simulink model "ANN_MultiLoad_Generated"  (R2023a)
settings: Solver=VariableStepAuto  StartTime=0.0  StopTime=10.0  RelTol=1e-3
libraries: neural x25
settings Model: Creator=Sooraj Mohan  LastModifiedBy=Sooraj Mohan

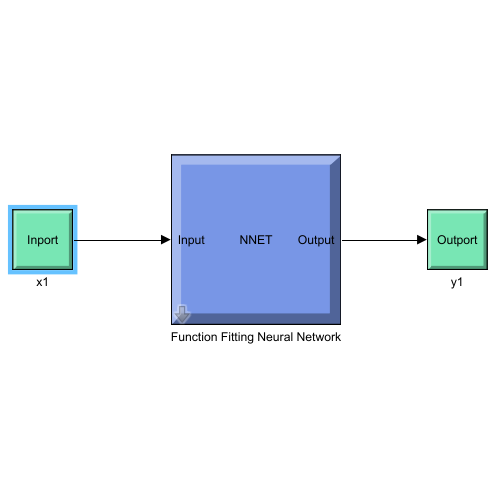
[thumbnail: Simulink's stored preview of the top-level diagram]
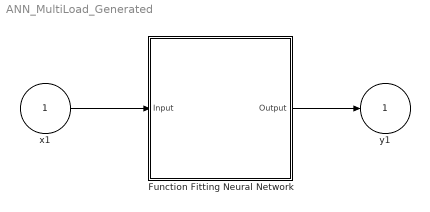
== system ANN_MultiLoad_Generated ==
  x1 : Inport  PortDimensions=3
      mask Display: e = 0.06;c1 = [120 230 180]/255;c2 = ([120 230 180]+0)/(256+128);c3 = ([120 230 180]+128)/(256+128);patch([0 1 1 0],[0 0 1 1],c1);patch([0 1 1 1-e 1-e 0+e],[0 0 1 1-e 0+e 0+e],c2);patch([0 0 1 1-e 0+e 0+e],[0 1 1 1-e 1-e 0+e],c3);plot([0 1 1 0 0],[0 0 1 1 0]);disp('Inport');
  Function Fitting Neural Network : Subsystem
      mask help: Function Fitting Neural Network
      mask Display: e = 0.06;c1 = [120 150 230]/255;c2 = ([120 150 230]+0)/383;c3 = ([120 150 230]+128)/383;patch([0 1 1 0],[0 0 1 1],c1);patch([0 1 1 1-e 1-e 0+e],[0 0 1 1-e 0+e 0+e],c2);patch([0 0 1 1-e 0+e 0+e],[0 1 1 1-e 1-e 0+e],c3);plot([0 1 1 0 0],[0 0 1 1 0]);fprintf('NNET');port_label('input',1,' Input');port_label('output',1,'Output ');
  y1 : Outport  PortDimensions=1
      mask Display: e = 0.06;c1 = [120 230 180]/255;c2 = ([120 230 180]+0)/(256+128);c3 = ([120 230 180]+128)/(256+128);patch([0 1 1 0],[0 0 1 1],c1);patch([0 1 1 1-e 1-e 0+e],[0 0 1 1-e 0+e 0+e],c2);patch([0 0 1 1-e 0+e 0+e],[0 1 1 1-e 1-e 0+e],c3);plot([0 1 1 0 0],[0 0 1 1 0]);disp('Outport');
  wires:
  x1/1 -> Function Fitting Neural Network/1(Input)
  Function Fitting Neural Network/1(Output) -> y1/1

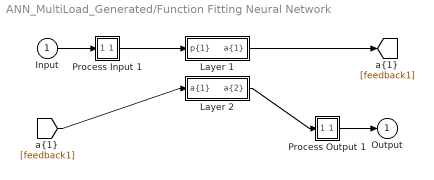
== system ANN_MultiLoad_Generated/Function Fitting Neural Network ==
  Input : Inport  PortDimensions=3
      mask Display: e = 0.06;c1 = [120 230 180]/255;c2 = ([120 230 180]+0)/(256+128);c3 = ([120 230 180]+128)/(256+128);patch([0 1 1 0],[0 0 1 1],c1);patch([0 1 1 1-e 1-e 0+e],[0 0 1 1-e 0+e 0+e],c2);patch([0 0 1 1-e 0+e 0+e],[0 1 1 1-e 1-e 0+e],c3);plot([0 1 1 0 0],[0 0 1 1 0]);
  Layer 1 : Subsystem
      mask Display: e = 0.06;c1 = [120 150 230]/255;c2 = ([120 150 230]+0)/383;c3 = ([120 150 230]+128)/383;patch([0 1 1 0],[0 0 1 1],c1);patch([0 1 1 1-e 1-e 0+e],[0 0 1 1-e 0+e 0+e],c2);patch([0 0 1 1-e 0+e 0+e],[0 1 1 1-e 1-e 0+e],c3);plot([0 1 1 0 0],[0 0 1 1 0]);
  Layer 2 : Subsystem
      mask Display: e = 0.06;c1 = [120 150 230]/255;c2 = ([120 150 230]+0)/383;c3 = ([120 150 230]+128)/383;patch([0 1 1 0],[0 0 1 1],c1);patch([0 1 1 1-e 1-e 0+e],[0 0 1 1-e 0+e 0+e],c2);patch([0 0 1 1-e 0+e 0+e],[0 1 1 1-e 1-e 0+e],c3);plot([0 1 1 0 0],[0 0 1 1 0]);
  Process Input 1 : Subsystem
      mask Display: e = 0.06;c1 = [120 150 230]/255;c2 = ([120 150 230]+0)/383;c3 = ([120 150 230]+128)/383;patch([0 1 1 0],[0 0 1 1],c1);patch([0 1 1 1-e 1-e 0+e],[0 0 1 1-e 0+e 0+e],c2);patch([0 0 1 1-e 0+e 0+e],[0 1 1 1-e 1-e 0+e],c3);plot([0 1 1 0 0],[0 0 1 1 0]);
  Process Output 1 : Subsystem
      mask Display: e = 0.06;c1 = [120 150 230]/255;c2 = ([120 150 230]+0)/383;c3 = ([120 150 230]+128)/383;patch([0 1 1 0],[0 0 1 1],c1);patch([0 1 1 1-e 1-e 0+e],[0 0 1 1-e 0+e 0+e],c2);patch([0 0 1 1-e 0+e 0+e],[0 1 1 1-e 1-e 0+e],c3);plot([0 1 1 0 0],[0 0 1 1 0]);
  Output : Outport  InitialOutput=0
      mask Display: e = 0.06;c1 = [120 230 180]/255;c2 = ([120 230 180]+0)/(256+128);c3 = ([120 230 180]+128)/(256+128);patch([0 1 1 0],[0 0 1 1],c1);patch([0 1 1 1-e 1-e 0+e],[0 0 1 1-e 0+e 0+e],c2);patch([0 0 1 1-e 0+e 0+e],[0 1 1 1-e 1-e 0+e],c3);plot([0 1 1 0 0],[0 0 1 1 0]);
  wires:
  Input/1 -> Process Input 1/1(x)
  Process Output 1/1(y) -> Output/1
  Process Input 1/1(p) -> Layer 1/1("p{1}")
  Layer 1/1("a{1}") -> [feedback1]
  [feedback1] -> Layer 2/1("a{1} ")
  Layer 2/1("a{2}") -> Process Output 1/1(a)

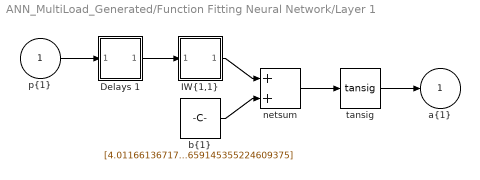
== system ANN_MultiLoad_Generated/Function Fitting Neural Network/Layer 1 ==
  "p{1}" : Inport  PortDimensions=3
      mask Display: e = 0.06;c1 = [120 230 180]/255;c2 = ([120 230 180]+0)/(256+128);c3 = ([120 230 180]+128)/(256+128);patch([0 1 1 0],[0 0 1 1],c1);patch([0 1 1 1-e 1-e 0+e],[0 0 1 1-e 0+e 0+e],c2);patch([0 0 1 1-e 0+e 0+e],[0 1 1 1-e 1-e 0+e],c3);plot([0 1 1 0 0],[0 0 1 1 0]);
  Delays 1 : Subsystem
      mask Display: e = 0.06;c1 = [120 150 230]/255;c2 = ([120 150 230]+0)/383;c3 = ([120 150 230]+128)/383;patch([0 1 1 0],[0 0 1 1],c1);patch([0 1 1 1-e 1-e 0+e],[0 0 1 1-e 0+e 0+e],c2);patch([0 0 1 1-e 0+e 0+e],[0 1 1 1-e 1-e 0+e],c3);plot([0 1 1 0 0],[0 0 1 1 0]);disp('0');
  "IW{1,1}" : Subsystem
      mask Display: e = 0.06;c1 = [120 150 230]/255;c2 = ([120 150 230]+0)/383;c3 = ([120 150 230]+128)/383;patch([0 1 1 0],[0 0 1 1],c1);patch([0 1 1 1-e 1-e 0+e],[0 0 1 1-e 0+e 0+e],c2);patch([0 0 1 1-e 0+e 0+e],[0 1 1 1-e 1-e 0+e],c3);plot([0 1 1 0 0],[0 0 1 1 0]);disp('W');
  "b{1}" : Constant  Value=[4.01166136717708976533458553603850305080413818359375;3.425657584804036925874015651061199605464935302734375;2.945133302338741376757980106049217283725738525390625;2.487472514834082826240546637563966214656829833984375;-2.198586640079299936445522689609788358211517333984375;-1.6511881060762032547017952310852706432342529296875;-0.9569310901758696363827993991435505449771881103515625;0.80526211729380448023363214815617538988590240478515625;0.63594565591895457767890320610604248940944671630859375;0.5017187841956556315636817089398391544818878173828125;0.09104143474311969519430220998401637189090251922607421875;-0.74022312093395414844820834332494996488094329833984375;-1.012970720944128544260820490308105945587158203125;-1.3663031771011218129530107034952379763126373291015625;1.8030354517322588758787560436758212745189666748046875;2.208400225146431861134033169946633279323577880859375;2.71632750565131431130794226191937923431396484375;-3.080179604871890131079226193833164870738983154296875;3.44002398306910261993607491604052484035491943359375;-3.78824406270324853807096587843261659145355224609375]
      mask Display: e = 0.06;c1 = [120 150 230]/255;c2 = ([120 150 230]+0)/383;c3 = ([120 150 230]+128)/383;patch([0 1 1 0],[0 0 1 1],c1);patch([0 1 1 1-e 1-e 0+e],[0 0 1 1-e 0+e 0+e],c2);patch([0 0 1 1-e 0+e 0+e],[0 1 1 1-e 1-e 0+e],c3);plot([0 1 1 0 0],[0 0 1 1 0]);disp('b');
  netsum : Sum  Inputs=2  InputSameDT=on  SaturateOnIntegerOverflow=on  OutDataTypeStr=Inherit: Same as first input
      mask Display: e = 0.06;c1 = [120 150 230]/255;c2 = ([120 150 230]+0)/383;c3 = ([120 150 230]+128)/383;patch([0 1 1 0],[0 0 1 1],c1);patch([0 1 1 1-e 1-e 0+e],[0 0 1 1-e 0+e 0+e],c2);patch([0 0 1 1-e 0+e 0+e],[0 1 1 1-e 1-e 0+e],c3);plot([0 1 1 0 0],[0 0 1 1 0]);disp('+');
  tansig : neural/Transfer Functions/tansig
  "a{1}" : Outport  InitialOutput=[0;0;0;0;0;0;0;0;0;0;0;0;0;0;0;0;0;0;0;0]
      mask Display: e = 0.06;c1 = [120 230 180]/255;c2 = ([120 230 180]+0)/(256+128);c3 = ([120 230 180]+128)/(256+128);patch([0 1 1 0],[0 0 1 1],c1);patch([0 1 1 1-e 1-e 0+e],[0 0 1 1-e 0+e 0+e],c2);patch([0 0 1 1-e 0+e 0+e],[0 1 1 1-e 1-e 0+e],c3);plot([0 1 1 0 0],[0 0 1 1 0]);
  wires:
  "p{1}"/1 -> Delays 1/1("p{1}")
  Delays 1/1("pd{1,1}") -> "IW{1,1}"/1("pd{1,1}")
  "IW{1,1}"/1("iz{1,1}") -> netsum/1
  "b{1}"/1 -> netsum/2
  netsum/1 -> tansig/1
  tansig/1 -> "a{1}"/1

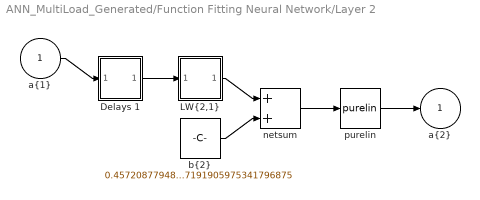
== system ANN_MultiLoad_Generated/Function Fitting Neural Network/Layer 2 ==
  "a{1} " : Inport  PortDimensions=20
      mask Display: e = 0.06;c1 = [120 230 180]/255;c2 = ([120 230 180]+0)/(256+128);c3 = ([120 230 180]+128)/(256+128);patch([0 1 1 0],[0 0 1 1],c1);patch([0 1 1 1-e 1-e 0+e],[0 0 1 1-e 0+e 0+e],c2);patch([0 0 1 1-e 0+e 0+e],[0 1 1 1-e 1-e 0+e],c3);plot([0 1 1 0 0],[0 0 1 1 0]);
  Delays 1 : Subsystem
      mask Display: e = 0.06;c1 = [120 150 230]/255;c2 = ([120 150 230]+0)/383;c3 = ([120 150 230]+128)/383;patch([0 1 1 0],[0 0 1 1],c1);patch([0 1 1 1-e 1-e 0+e],[0 0 1 1-e 0+e 0+e],c2);patch([0 0 1 1-e 0+e 0+e],[0 1 1 1-e 1-e 0+e],c3);plot([0 1 1 0 0],[0 0 1 1 0]);disp('0');
  "LW{2,1}" : Subsystem
      mask Display: e = 0.06;c1 = [120 150 230]/255;c2 = ([120 150 230]+0)/383;c3 = ([120 150 230]+128)/383;patch([0 1 1 0],[0 0 1 1],c1);patch([0 1 1 1-e 1-e 0+e],[0 0 1 1-e 0+e 0+e],c2);patch([0 0 1 1-e 0+e 0+e],[0 1 1 1-e 1-e 0+e],c3);plot([0 1 1 0 0],[0 0 1 1 0]);disp('W');
  "b{2}" : Constant  Value=0.4572087794873869182055159399169497191905975341796875
      mask Display: e = 0.06;c1 = [120 150 230]/255;c2 = ([120 150 230]+0)/383;c3 = ([120 150 230]+128)/383;patch([0 1 1 0],[0 0 1 1],c1);patch([0 1 1 1-e 1-e 0+e],[0 0 1 1-e 0+e 0+e],c2);patch([0 0 1 1-e 0+e 0+e],[0 1 1 1-e 1-e 0+e],c3);plot([0 1 1 0 0],[0 0 1 1 0]);disp('b');
  netsum : Sum  Inputs=2  InputSameDT=on  SaturateOnIntegerOverflow=on  OutDataTypeStr=Inherit: Same as first input
      mask Display: e = 0.06;c1 = [120 150 230]/255;c2 = ([120 150 230]+0)/383;c3 = ([120 150 230]+128)/383;patch([0 1 1 0],[0 0 1 1],c1);patch([0 1 1 1-e 1-e 0+e],[0 0 1 1-e 0+e 0+e],c2);patch([0 0 1 1-e 0+e 0+e],[0 1 1 1-e 1-e 0+e],c3);plot([0 1 1 0 0],[0 0 1 1 0]);disp('+');
  purelin : neural/Transfer Functions/purelin
  "a{2}" : Outport  InitialOutput=0
      mask Display: e = 0.06;c1 = [120 230 180]/255;c2 = ([120 230 180]+0)/(256+128);c3 = ([120 230 180]+128)/(256+128);patch([0 1 1 0],[0 0 1 1],c1);patch([0 1 1 1-e 1-e 0+e],[0 0 1 1-e 0+e 0+e],c2);patch([0 0 1 1-e 0+e 0+e],[0 1 1 1-e 1-e 0+e],c3);plot([0 1 1 0 0],[0 0 1 1 0]);
  wires:
  "a{1} "/1 -> Delays 1/1("p{2}")
  Delays 1/1("pd{2,1}") -> "LW{2,1}"/1("ad{2,1}")
  "LW{2,1}"/1("lz{2,1}") -> netsum/1
  "b{2}"/1 -> netsum/2
  netsum/1 -> purelin/1
  purelin/1 -> "a{2}"/1

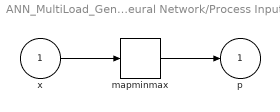
== system ANN_MultiLoad_Generated/Function Fitting Neural Network/Process Input 1 ==
  x : Inport  PortDimensions=3
      mask Display: e = 0.06;c1 = [120 230 180]/255;c2 = ([120 230 180]+0)/(256+128);c3 = ([120 230 180]+128)/(256+128);patch([0 1 1 0],[0 0 1 1],c1);patch([0 1 1 1-e 1-e 0+e],[0 0 1 1-e 0+e 0+e],c2);patch([0 0 1 1-e 0+e 0+e],[0 1 1 1-e 1-e 0+e],c3);plot([0 1 1 0 0],[0 0 1 1 0]);
  mapminmax : neural/Processing Functions/mapminmax  xmin=[-5.41533881963086471955648448784;-353.856954219733665922831278294;400.000000000000056843418860808]  xmax=[5.40694529891772912577607712592;355.597694951485948422487126663;400.000000000000113686837721616]  ymin=-1  ymax=1
  p : Outport  PortDimensions=3
      mask Display: e = 0.06;c1 = [120 230 180]/255;c2 = ([120 230 180]+0)/(256+128);c3 = ([120 230 180]+128)/(256+128);patch([0 1 1 0],[0 0 1 1],c1);patch([0 1 1 1-e 1-e 0+e],[0 0 1 1-e 0+e 0+e],c2);patch([0 0 1 1-e 0+e 0+e],[0 1 1 1-e 1-e 0+e],c3);plot([0 1 1 0 0],[0 0 1 1 0]);
  wires:
  x/1 -> mapminmax/1
  mapminmax/1 -> p/1

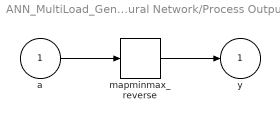
== system ANN_MultiLoad_Generated/Function Fitting Neural Network/Process Output 1 ==
  a : Inport  PortDimensions=1
      mask Display: e = 0.06;c1 = [120 230 180]/255;c2 = ([120 230 180]+0)/(256+128);c3 = ([120 230 180]+128)/(256+128);patch([0 1 1 0],[0 0 1 1],c1);patch([0 1 1 1-e 1-e 0+e],[0 0 1 1-e 0+e 0+e],c2);patch([0 0 1 1-e 0+e 0+e],[0 1 1 1-e 1-e 0+e],c3);plot([0 1 1 0 0],[0 0 1 1 0]);
  mapminmax_reverse : neural/Processing Functions/mapminmax_reverse  xmin=-85.1861603832918632406290271319  xmax=79.5292501519603263204771792516  ymin=-1  ymax=1
  y : Outport  PortDimensions=1
      mask Display: e = 0.06;c1 = [120 230 180]/255;c2 = ([120 230 180]+0)/(256+128);c3 = ([120 230 180]+128)/(256+128);patch([0 1 1 0],[0 0 1 1],c1);patch([0 1 1 1-e 1-e 0+e],[0 0 1 1-e 0+e 0+e],c2);patch([0 0 1 1-e 0+e 0+e],[0 1 1 1-e 1-e 0+e],c3);plot([0 1 1 0 0],[0 0 1 1 0]);
  wires:
  a/1 -> mapminmax_reverse/1
  mapminmax_reverse/1 -> y/1

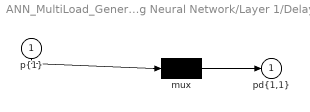
== system ANN_MultiLoad_Generated/Function Fitting Neural Network/Layer 1/Delays 1 ==
  "p{1}" : Inport  PortDimensions=3
      mask Display: e = 0.06;c1 = [120 230 180]/255;c2 = ([120 230 180]+0)/(256+128);c3 = ([120 230 180]+128)/(256+128);patch([0 1 1 0],[0 0 1 1],c1);patch([0 1 1 1-e 1-e 0+e],[0 0 1 1-e 0+e 0+e],c2);patch([0 0 1 1-e 0+e 0+e],[0 1 1 1-e 1-e 0+e],c3);plot([0 1 1 0 0],[0 0 1 1 0]);
  mux : Mux  Inputs=1
      mask Display: e = 0.06;c1 = [120 150 230]/255;c2 = ([120 150 230]+0)/383;c3 = ([120 150 230]+128)/383;patch([0 1 1 0],[0 0 1 1],c1);patch([0 1 1 1-e 1-e 0+e],[0 0 1 1-e 0+e 0+e],c2);patch([0 0 1 1-e 0+e 0+e],[0 1 1 1-e 1-e 0+e],c3);plot([0 1 1 0 0],[0 0 1 1 0]);disp('Mux')
  "pd{1,1}" : Outport
      mask Display: e = 0.06;c1 = [120 230 180]/255;c2 = ([120 230 180]+0)/(256+128);c3 = ([120 230 180]+128)/(256+128);patch([0 1 1 0],[0 0 1 1],c1);patch([0 1 1 1-e 1-e 0+e],[0 0 1 1-e 0+e 0+e],c2);patch([0 0 1 1-e 0+e 0+e],[0 1 1 1-e 1-e 0+e],c3);plot([0 1 1 0 0],[0 0 1 1 0]);
  wires:
  "p{1}"/1 -> mux/1
  mux/1 -> "pd{1,1}"/1

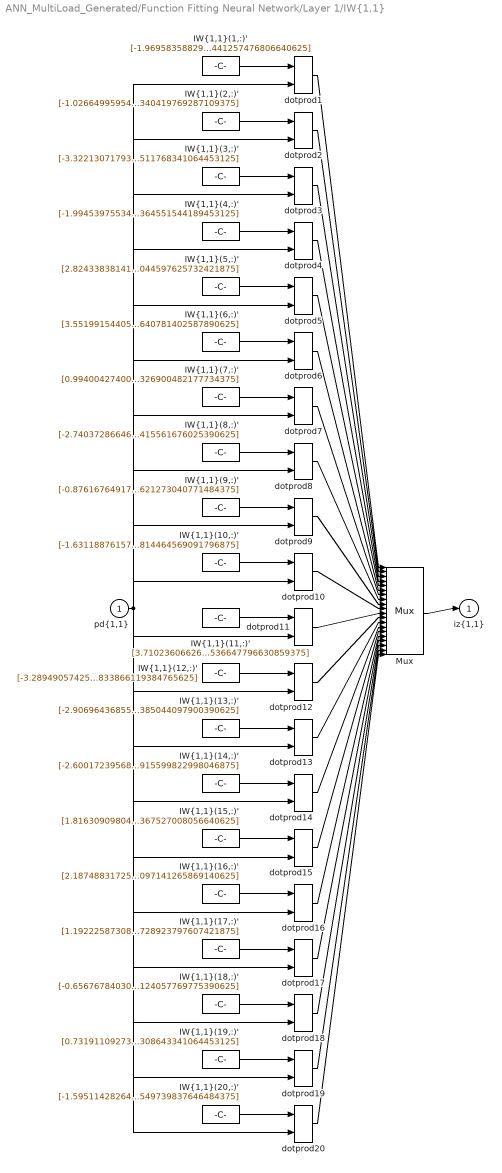
== system ANN_MultiLoad_Generated/Function Fitting Neural Network/Layer 1/IW{1,1} ==
  "pd{1,1}" : Inport  PortDimensions=3
      mask Display: e = 0.06;c1 = [120 230 180]/255;c2 = ([120 230 180]+0)/(256+128);c3 = ([120 230 180]+128)/(256+128);patch([0 1 1 0],[0 0 1 1],c1);patch([0 1 1 1-e 1-e 0+e],[0 0 1 1-e 0+e 0+e],c2);patch([0 0 1 1-e 0+e 0+e],[0 1 1 1-e 1-e 0+e],c3);plot([0 1 1 0 0],[0 0 1 1 0]);
  "IW{1,1}(1,:)'" : Constant  Value=[-1.96958358829980539894677349366247653961181640625;1.918521251483812140037343851872719824314117431640625;2.29210042612150033392026671208441257476806640625]
      mask Display: e = 0.06;c1 = [120 150 230]/255;c2 = ([120 150 230]+0)/383;c3 = ([120 150 230]+128)/383;patch([0 1 1 0],[0 0 1 1],c1);patch([0 1 1 1-e 1-e 0+e],[0 0 1 1-e 0+e 0+e],c2);patch([0 0 1 1-e 0+e 0+e],[0 1 1 1-e 1-e 0+e],c3);plot([0 1 1 0 0],[0 0 1 1 0]);disp('Weights');
  "IW{1,1}(10,:)'" : Constant  Value=[-1.6311887615787288297042323392815887928009033203125;2.51590885704565447866798422182910144329071044921875;-2.3411727844511727170129233854822814464569091796875]
      mask Display: e = 0.06;c1 = [120 150 230]/255;c2 = ([120 150 230]+0)/383;c3 = ([120 150 230]+128)/383;patch([0 1 1 0],[0 0 1 1],c1);patch([0 1 1 1-e 1-e 0+e],[0 0 1 1-e 0+e 0+e],c2);patch([0 0 1 1-e 0+e 0+e],[0 1 1 1-e 1-e 0+e],c3);plot([0 1 1 0 0],[0 0 1 1 0]);disp('Weights');
  "IW{1,1}(11,:)'" : Constant  Value=[3.71023606626158386490033080917783081531524658203125;-0.5979197475541944140076111580128781497478485107421875;-0.2575045382185476849912220131955109536647796630859375]
      mask Display: e = 0.06;c1 = [120 150 230]/255;c2 = ([120 150 230]+0)/383;c3 = ([120 150 230]+128)/383;patch([0 1 1 0],[0 0 1 1],c1);patch([0 1 1 1-e 1-e 0+e],[0 0 1 1-e 0+e 0+e],c2);patch([0 0 1 1-e 0+e 0+e],[0 1 1 1-e 1-e 0+e],c3);plot([0 1 1 0 0],[0 0 1 1 0]);disp('Weights');
  "IW{1,1}(12,:)'" : Constant  Value=[-3.289490574255142352200209643342532217502593994140625;-0.5469995320266207716741746480693109333515167236328125;-1.6949446183999461457148072440759278833866119384765625]
      mask Display: e = 0.06;c1 = [120 150 230]/255;c2 = ([120 150 230]+0)/383;c3 = ([120 150 230]+128)/383;patch([0 1 1 0],[0 0 1 1],c1);patch([0 1 1 1-e 1-e 0+e],[0 0 1 1-e 0+e 0+e],c2);patch([0 0 1 1-e 0+e 0+e],[0 1 1 1-e 1-e 0+e],c3);plot([0 1 1 0 0],[0 0 1 1 0]);disp('Weights');
  "IW{1,1}(13,:)'" : Constant  Value=[-2.906964368554389555043826476321555674076080322265625;-0.5995612852190375097194419140578247606754302978515625;2.299154545812025052242688616388477385044097900390625]
      mask Display: e = 0.06;c1 = [120 150 230]/255;c2 = ([120 150 230]+0)/383;c3 = ([120 150 230]+128)/383;patch([0 1 1 0],[0 0 1 1],c1);patch([0 1 1 1-e 1-e 0+e],[0 0 1 1-e 0+e 0+e],c2);patch([0 0 1 1-e 0+e 0+e],[0 1 1 1-e 1-e 0+e],c3);plot([0 1 1 0 0],[0 0 1 1 0]);disp('Weights');
  "IW{1,1}(14,:)'" : Constant  Value=[-2.60017239568569547003562547615729272365570068359375;-1.2913554073851207792955619879649020731449127197265625;-2.40019667610683296032902944716624915599822998046875]
      mask Display: e = 0.06;c1 = [120 150 230]/255;c2 = ([120 150 230]+0)/383;c3 = ([120 150 230]+128)/383;patch([0 1 1 0],[0 0 1 1],c1);patch([0 1 1 1-e 1-e 0+e],[0 0 1 1-e 0+e 0+e],c2);patch([0 0 1 1-e 0+e 0+e],[0 1 1 1-e 1-e 0+e],c3);plot([0 1 1 0 0],[0 0 1 1 0]);disp('Weights');
  "IW{1,1}(15,:)'" : Constant  Value=[1.8163090980494087656182955470285378396511077880859375;0.1027208588357631235954414705702220089733600616455078125;-3.33268860031713476388404160388745367527008056640625]
      mask Display: e = 0.06;c1 = [120 150 230]/255;c2 = ([120 150 230]+0)/383;c3 = ([120 150 230]+128)/383;patch([0 1 1 0],[0 0 1 1],c1);patch([0 1 1 1-e 1-e 0+e],[0 0 1 1-e 0+e 0+e],c2);patch([0 0 1 1-e 0+e 0+e],[0 1 1 1-e 1-e 0+e],c3);plot([0 1 1 0 0],[0 0 1 1 0]);disp('Weights');
  "IW{1,1}(16,:)'" : Constant  Value=[2.18748831725833259298497068812139332294464111328125;0.10090970176754243681216394179500639438629150390625;-3.0963102908207762453685063519515097141265869140625]
      mask Display: e = 0.06;c1 = [120 150 230]/255;c2 = ([120 150 230]+0)/383;c3 = ([120 150 230]+128)/383;patch([0 1 1 0],[0 0 1 1],c1);patch([0 1 1 1-e 1-e 0+e],[0 0 1 1-e 0+e 0+e],c2);patch([0 0 1 1-e 0+e 0+e],[0 1 1 1-e 1-e 0+e],c3);plot([0 1 1 0 0],[0 0 1 1 0]);disp('Weights');
  "IW{1,1}(17,:)'" : Constant  Value=[1.19222587308537786299211802543140947818756103515625;2.60340339909535156692754753748886287212371826171875;-2.433568542835882198005492682568728923797607421875]
      mask Display: e = 0.06;c1 = [120 150 230]/255;c2 = ([120 150 230]+0)/383;c3 = ([120 150 230]+128)/383;patch([0 1 1 0],[0 0 1 1],c1);patch([0 1 1 1-e 1-e 0+e],[0 0 1 1-e 0+e 0+e],c2);patch([0 0 1 1-e 0+e 0+e],[0 1 1 1-e 1-e 0+e],c3);plot([0 1 1 0 0],[0 0 1 1 0]);disp('Weights');
  "IW{1,1}(18,:)'" : Constant  Value=[-0.65676784030766033328774256005999632179737091064453125;3.60318263358925516826047896756790578365325927734375;-0.7192382964292927116645159912877716124057769775390625]
      mask Display: e = 0.06;c1 = [120 150 230]/255;c2 = ([120 150 230]+0)/383;c3 = ([120 150 230]+128)/383;patch([0 1 1 0],[0 0 1 1],c1);patch([0 1 1 1-e 1-e 0+e],[0 0 1 1-e 0+e 0+e],c2);patch([0 0 1 1-e 0+e 0+e],[0 1 1 1-e 1-e 0+e],c3);plot([0 1 1 0 0],[0 0 1 1 0]);disp('Weights');
  "IW{1,1}(19,:)'" : Constant  Value=[0.73191109273039334226496066548861563205718994140625;2.25441141521850685336403330438770353794097900390625;-2.93828389411340840098318949458189308643341064453125]
      mask Display: e = 0.06;c1 = [120 150 230]/255;c2 = ([120 150 230]+0)/383;c3 = ([120 150 230]+128)/383;patch([0 1 1 0],[0 0 1 1],c1);patch([0 1 1 1-e 1-e 0+e],[0 0 1 1-e 0+e 0+e],c2);patch([0 0 1 1-e 0+e 0+e],[0 1 1 1-e 1-e 0+e],c3);plot([0 1 1 0 0],[0 0 1 1 0]);disp('Weights');
  "IW{1,1}(2,:)'" : Constant  Value=[-1.0266499595402311939551509567536413669586181640625;-3.750127303457734040392779206740669906139373779296875;0.3558927058893279760098948827362619340419769287109375]
      mask Display: e = 0.06;c1 = [120 150 230]/255;c2 = ([120 150 230]+0)/383;c3 = ([120 150 230]+128)/383;patch([0 1 1 0],[0 0 1 1],c1);patch([0 1 1 1-e 1-e 0+e],[0 0 1 1-e 0+e 0+e],c2);patch([0 0 1 1-e 0+e 0+e],[0 1 1 1-e 1-e 0+e],c3);plot([0 1 1 0 0],[0 0 1 1 0]);disp('Weights');
  "IW{1,1}(20,:)'" : Constant  Value=[-1.59511428264959054246219238848425447940826416015625;-0.950804370965463885312374259228818118572235107421875;3.32740866167332427494329749606549739837646484375]
      mask Display: e = 0.06;c1 = [120 150 230]/255;c2 = ([120 150 230]+0)/383;c3 = ([120 150 230]+128)/383;patch([0 1 1 0],[0 0 1 1],c1);patch([0 1 1 1-e 1-e 0+e],[0 0 1 1-e 0+e 0+e],c2);patch([0 0 1 1-e 0+e 0+e],[0 1 1 1-e 1-e 0+e],c3);plot([0 1 1 0 0],[0 0 1 1 0]);disp('Weights');
  "IW{1,1}(3,:)'" : Constant  Value=[-3.3221307179311754254058541846461594104766845703125;1.470211676342646267556801831233315169811248779296875;-1.160407496704341401283500090357847511768341064453125]
      mask Display: e = 0.06;c1 = [120 150 230]/255;c2 = ([120 150 230]+0)/383;c3 = ([120 150 230]+128)/383;patch([0 1 1 0],[0 0 1 1],c1);patch([0 1 1 1-e 1-e 0+e],[0 0 1 1-e 0+e 0+e],c2);patch([0 0 1 1-e 0+e 0+e],[0 1 1 1-e 1-e 0+e],c3);plot([0 1 1 0 0],[0 0 1 1 0]);disp('Weights');
  "IW{1,1}(4,:)'" : Constant  Value=[-1.9945397553436254867165189352817833423614501953125;-1.2838945124631575556151119599235244095325469970703125;2.661710597616452123048702560481615364551544189453125]
      mask Display: e = 0.06;c1 = [120 150 230]/255;c2 = ([120 150 230]+0)/383;c3 = ([120 150 230]+128)/383;patch([0 1 1 0],[0 0 1 1],c1);patch([0 1 1 1-e 1-e 0+e],[0 0 1 1-e 0+e 0+e],c2);patch([0 0 1 1-e 0+e 0+e],[0 1 1 1-e 1-e 0+e],c3);plot([0 1 1 0 0],[0 0 1 1 0]);disp('Weights');
  "IW{1,1}(5,:)'" : Constant  Value=[2.824338381411645837459900576504878699779510498046875;-0.8391692684293392545669121318496763706207275390625;2.400397949837205668899287047679536044597625732421875]
      mask Display: e = 0.06;c1 = [120 150 230]/255;c2 = ([120 150 230]+0)/383;c3 = ([120 150 230]+128)/383;patch([0 1 1 0],[0 0 1 1],c1);patch([0 1 1 1-e 1-e 0+e],[0 0 1 1-e 0+e 0+e],c2);patch([0 0 1 1-e 0+e 0+e],[0 1 1 1-e 1-e 0+e],c3);plot([0 1 1 0 0],[0 0 1 1 0]);disp('Weights');
  "IW{1,1}(6,:)'" : Constant  Value=[3.551991544055625116271812657942064106464385986328125;1.1022017018245733321890611478011123836040496826171875;0.25867677418343115736121262671076692640781402587890625]
      mask Display: e = 0.06;c1 = [120 150 230]/255;c2 = ([120 150 230]+0)/383;c3 = ([120 150 230]+128)/383;patch([0 1 1 0],[0 0 1 1],c1);patch([0 1 1 1-e 1-e 0+e],[0 0 1 1-e 0+e 0+e],c2);patch([0 0 1 1-e 0+e 0+e],[0 1 1 1-e 1-e 0+e],c3);plot([0 1 1 0 0],[0 0 1 1 0]);disp('Weights');
  "IW{1,1}(7,:)'" : Constant  Value=[0.9940042740010686106444381948676891624927520751953125;3.647901481936774548131552364793606102466583251953125;1.0563202763403347628212713971151970326900482177734375]
      mask Display: e = 0.06;c1 = [120 150 230]/255;c2 = ([120 150 230]+0)/383;c3 = ([120 150 230]+128)/383;patch([0 1 1 0],[0 0 1 1],c1);patch([0 1 1 1-e 1-e 0+e],[0 0 1 1-e 0+e 0+e],c2);patch([0 0 1 1-e 0+e 0+e],[0 1 1 1-e 1-e 0+e],c3);plot([0 1 1 0 0],[0 0 1 1 0]);disp('Weights');
  "IW{1,1}(8,:)'" : Constant  Value=[-2.74037286646862465744334258488379418849945068359375;-3.116088599926580826604549656622111797332763671875;0.7371387791378902765160319177084602415561676025390625]
      mask Display: e = 0.06;c1 = [120 150 230]/255;c2 = ([120 150 230]+0)/383;c3 = ([120 150 230]+128)/383;patch([0 1 1 0],[0 0 1 1],c1);patch([0 1 1 1-e 1-e 0+e],[0 0 1 1-e 0+e 0+e],c2);patch([0 0 1 1-e 0+e 0+e],[0 1 1 1-e 1-e 0+e],c3);plot([0 1 1 0 0],[0 0 1 1 0]);disp('Weights');
  "IW{1,1}(9,:)'" : Constant  Value=[-0.87616764917543010771083800136693753302097320556640625;3.4095142218128220434891773038543760776519775390625;-1.9511939532637272431969677199958823621273040771484375]
      mask Display: e = 0.06;c1 = [120 150 230]/255;c2 = ([120 150 230]+0)/383;c3 = ([120 150 230]+128)/383;patch([0 1 1 0],[0 0 1 1],c1);patch([0 1 1 1-e 1-e 0+e],[0 0 1 1-e 0+e 0+e],c2);patch([0 0 1 1-e 0+e 0+e],[0 1 1 1-e 1-e 0+e],c3);plot([0 1 1 0 0],[0 0 1 1 0]);disp('Weights');
  Mux : Mux  Inputs=20
      mask Display: e = 0.06;c1 = [120 150 230]/255;c2 = ([120 150 230]+0)/383;c3 = ([120 150 230]+128)/383;patch([0 1 1 0],[0 0 1 1],c1);patch([0 1 1 1-e 1-e 0+e],[0 0 1 1-e 0+e 0+e],c2);patch([0 0 1 1-e 0+e 0+e],[0 1 1 1-e 1-e 0+e],c3);plot([0 1 1 0 0],[0 0 1 1 0]);disp('Mux');
  dotprod{1..20} (20 alike) : neural/Weight Functions/dotprod
  "iz{1,1}" : Outport
      mask Display: e = 0.06;c1 = [120 230 180]/255;c2 = ([120 230 180]+0)/(256+128);c3 = ([120 230 180]+128)/(256+128);patch([0 1 1 0],[0 0 1 1],c1);patch([0 1 1 1-e 1-e 0+e],[0 0 1 1-e 0+e 0+e],c2);patch([0 0 1 1-e 0+e 0+e],[0 1 1 1-e 1-e 0+e],c3);plot([0 1 1 0 0],[0 0 1 1 0]);
  wires:
  "IW{1,1}(1,:)'"/1 -> dotprod1/1
  "pd{1,1}"/1 -> dotprod1/2, dotprod2/2, dotprod3/2, dotprod4/2, dotprod5/2, dotprod6/2, dotprod7/2, dotprod8/2, dotprod9/2, dotprod10/2, dotprod11/2, dotprod12/2, dotprod13/2, dotprod14/2, dotprod15/2, dotprod16/2, dotprod17/2, dotprod18/2, dotprod19/2, dotprod20/2
  dotprod1/1 -> Mux/1
  "IW{1,1}(2,:)'"/1 -> dotprod2/1
  dotprod2/1 -> Mux/2
  "IW{1,1}(3,:)'"/1 -> dotprod3/1
  dotprod3/1 -> Mux/3
  "IW{1,1}(4,:)'"/1 -> dotprod4/1
  dotprod4/1 -> Mux/4
  "IW{1,1}(5,:)'"/1 -> dotprod5/1
  dotprod5/1 -> Mux/5
  "IW{1,1}(6,:)'"/1 -> dotprod6/1
  dotprod6/1 -> Mux/6
  "IW{1,1}(7,:)'"/1 -> dotprod7/1
  dotprod7/1 -> Mux/7
  "IW{1,1}(8,:)'"/1 -> dotprod8/1
  dotprod8/1 -> Mux/8
  "IW{1,1}(9,:)'"/1 -> dotprod9/1
  dotprod9/1 -> Mux/9
  "IW{1,1}(10,:)'"/1 -> dotprod10/1
  dotprod10/1 -> Mux/10
  "IW{1,1}(11,:)'"/1 -> dotprod11/1
  dotprod11/1 -> Mux/11
  "IW{1,1}(12,:)'"/1 -> dotprod12/1
  dotprod12/1 -> Mux/12
  "IW{1,1}(13,:)'"/1 -> dotprod13/1
  dotprod13/1 -> Mux/13
  "IW{1,1}(14,:)'"/1 -> dotprod14/1
  dotprod14/1 -> Mux/14
  "IW{1,1}(15,:)'"/1 -> dotprod15/1
  dotprod15/1 -> Mux/15
  "IW{1,1}(16,:)'"/1 -> dotprod16/1
  dotprod16/1 -> Mux/16
  "IW{1,1}(17,:)'"/1 -> dotprod17/1
  dotprod17/1 -> Mux/17
  "IW{1,1}(18,:)'"/1 -> dotprod18/1
  dotprod18/1 -> Mux/18
  "IW{1,1}(19,:)'"/1 -> dotprod19/1
  dotprod19/1 -> Mux/19
  "IW{1,1}(20,:)'"/1 -> dotprod20/1
  dotprod20/1 -> Mux/20
  Mux/1 -> "iz{1,1}"/1

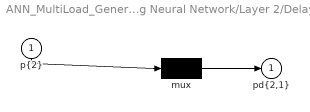
== system ANN_MultiLoad_Generated/Function Fitting Neural Network/Layer 2/Delays 1 ==
  "p{2}" : Inport  PortDimensions=20
      mask Display: e = 0.06;c1 = [120 230 180]/255;c2 = ([120 230 180]+0)/(256+128);c3 = ([120 230 180]+128)/(256+128);patch([0 1 1 0],[0 0 1 1],c1);patch([0 1 1 1-e 1-e 0+e],[0 0 1 1-e 0+e 0+e],c2);patch([0 0 1 1-e 0+e 0+e],[0 1 1 1-e 1-e 0+e],c3);plot([0 1 1 0 0],[0 0 1 1 0]);
  mux : Mux  Inputs=1
      mask Display: e = 0.06;c1 = [120 150 230]/255;c2 = ([120 150 230]+0)/383;c3 = ([120 150 230]+128)/383;patch([0 1 1 0],[0 0 1 1],c1);patch([0 1 1 1-e 1-e 0+e],[0 0 1 1-e 0+e 0+e],c2);patch([0 0 1 1-e 0+e 0+e],[0 1 1 1-e 1-e 0+e],c3);plot([0 1 1 0 0],[0 0 1 1 0]);disp('Mux')
  "pd{2,1}" : Outport
      mask Display: e = 0.06;c1 = [120 230 180]/255;c2 = ([120 230 180]+0)/(256+128);c3 = ([120 230 180]+128)/(256+128);patch([0 1 1 0],[0 0 1 1],c1);patch([0 1 1 1-e 1-e 0+e],[0 0 1 1-e 0+e 0+e],c2);patch([0 0 1 1-e 0+e 0+e],[0 1 1 1-e 1-e 0+e],c3);plot([0 1 1 0 0],[0 0 1 1 0]);
  wires:
  "p{2}"/1 -> mux/1
  mux/1 -> "pd{2,1}"/1

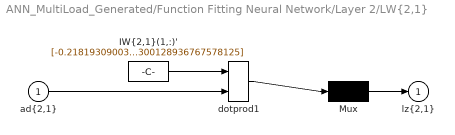
== system ANN_MultiLoad_Generated/Function Fitting Neural Network/Layer 2/LW{2,1} ==
  "ad{2,1}" : Inport  PortDimensions=20
      mask Display: e = 0.06;c1 = [120 230 180]/255;c2 = ([120 230 180]+0)/(256+128);c3 = ([120 230 180]+128)/(256+128);patch([0 1 1 0],[0 0 1 1],c1);patch([0 1 1 1-e 1-e 0+e],[0 0 1 1-e 0+e 0+e],c2);patch([0 0 1 1-e 0+e 0+e],[0 1 1 1-e 1-e 0+e],c3);plot([0 1 1 0 0],[0 0 1 1 0]);
  "IW{2,1}(1,:)'" : Constant  Value=[-0.2181930900351575497442269124803715385496616363525390625;-0.71401083996674519216441012758878059685230255126953125;0.7053305494279504817001225092099048197269439697265625;1.0915585642703486968230208731256425380706787109375;-0.04553528080116474308081109256818308494985103607177734375;-0.057166657961121032649476347842210088856518268585205078125;-0.55182568393647046800509770037024281919002532958984375;-0.9754616043134216596399710397236049175262451171875;0.815918636724976664709174656309187412261962890625;-0.04557498307649750224346263394181733019649982452392578125;0.2053493059552899679953696931988815777003765106201171875;0.254153507659776456417688450528657995164394378662109375;-0.305008776149595706161932184841134585440158843994140625;-0.31621814359051014786672340051154606044292449951171875;-0.473686437519729997003281596335000358521938323974609375;-0.437947730459071038477958381918142549693584442138671875;0.04284536460033894211818505937117151916027069091796875;0.22490992958266164958303079401957802474498748779296875;-0.945575217883591445655611096299253404140472412109375;-0.353035396197976247822936102238600142300128936767578125]
      mask Display: e = 0.06;c1 = [120 150 230]/255;c2 = ([120 150 230]+0)/383;c3 = ([120 150 230]+128)/383;patch([0 1 1 0],[0 0 1 1],c1);patch([0 1 1 1-e 1-e 0+e],[0 0 1 1-e 0+e 0+e],c2);patch([0 0 1 1-e 0+e 0+e],[0 1 1 1-e 1-e 0+e],c3);plot([0 1 1 0 0],[0 0 1 1 0]);disp('weights');
  Mux : Mux  Inputs=1
      mask Display: e = 0.06;c1 = [120 150 230]/255;c2 = ([120 150 230]+0)/383;c3 = ([120 150 230]+128)/383;patch([0 1 1 0],[0 0 1 1],c1);patch([0 1 1 1-e 1-e 0+e],[0 0 1 1-e 0+e 0+e],c2);patch([0 0 1 1-e 0+e 0+e],[0 1 1 1-e 1-e 0+e],c3);plot([0 1 1 0 0],[0 0 1 1 0]);disp('Mux');
  dotprod1 : neural/Weight Functions/dotprod
  "lz{2,1}" : Outport
      mask Display: e = 0.06;c1 = [120 230 180]/255;c2 = ([120 230 180]+0)/(256+128);c3 = ([120 230 180]+128)/(256+128);patch([0 1 1 0],[0 0 1 1],c1);patch([0 1 1 1-e 1-e 0+e],[0 0 1 1-e 0+e 0+e],c2);patch([0 0 1 1-e 0+e 0+e],[0 1 1 1-e 1-e 0+e],c3);plot([0 1 1 0 0],[0 0 1 1 0]);
  wires:
  "IW{2,1}(1,:)'"/1 -> dotprod1/1
  "ad{2,1}"/1 -> dotprod1/2
  dotprod1/1 -> Mux/1
  Mux/1 -> "lz{2,1}"/1
